simulink model "stewart_platform_model"  (R2020a)
settings: Solver=ode45  StartTime=0.0  StopTime=0.1  FixedStep=1e-4  MaxStep=0.2  RelTol=1e-4  AbsTol=1e-4
values from neighbouring files (symbols this model uses):
  ground = initializeGround('type', 'none')    [active_damping_dvf.m]    (also in active_damping_iff.m; active_damping_inertial.m; cubic_conf_coupling_cartesianl.m; cubic_conf_coupling_strutsl.m)
  payload = initializePayload('type', 'none')    [active_damping_dvf.m]    (also in active_damping_iff.m; active_damping_inertial.m; cubic_conf_coupling_cartesianl.m; cubic_conf_coupling_strutsl.m)
  s = zpk('s')    [active_damping_dvf.m]    (also in active_damping_iff.m; active_damping_inertial.m; cubic_conf_above_platforml.m; cubic_conf_coupling_cartesianl.m)
undefined symbols (not defined in the file or in its folder): X, Y, Z
libraries: sm_lib x29, nesl_utility x27, cstblocks x10
(part 1 of 2)
settings Model: Creator=thomas  LastModifiedBy=thomas
settings SolverCC: AutoScaleAbsTol=off
settings DataIOCC: SaveOutput=off  SignalLogging=off  DSMLogging=off  SaveTime=off  ReturnWorkspaceOutputs=off
settings DebuggingCC: SymbolicDimsDataTypeCodeGenerationDiagnostic=none
settings SFSimCC: CustomCodeUndefinedFunction=UseInterfaceOnly
settings SimscapeCC: SimscapeLogType=all  SimscapeLogSimulationStatistics=on  SimscapeLogDataHistory=10000
settings DiagnosticsConfigSet: SimMechanicsRigidlyBoundBlock=warning  SimMechanicsJointTargetOverSpecification=warning

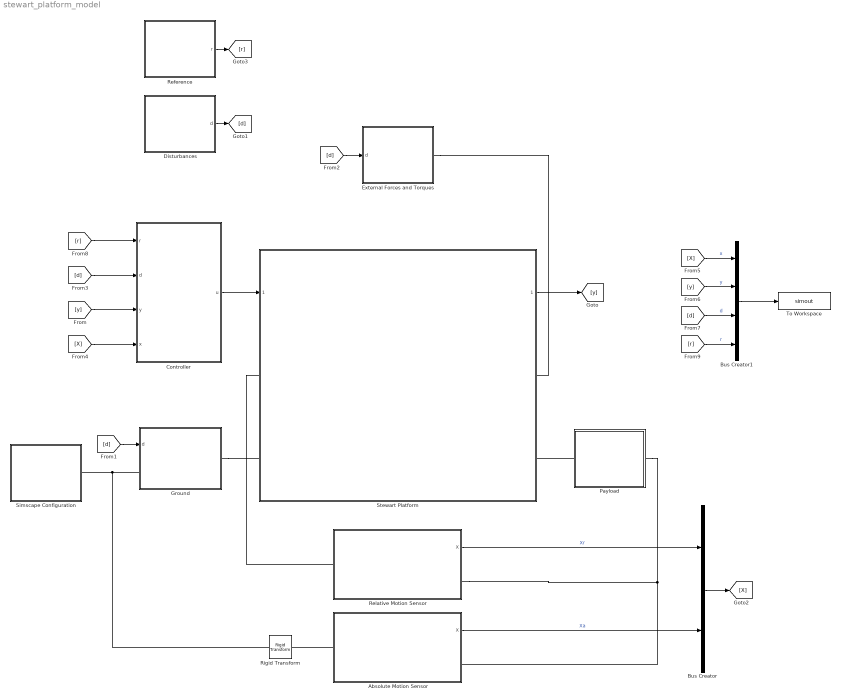
== system stewart_platform_model ==
  Absolute Motion Sensor : Subsystem
  Bus Creator : BusCreator  Inputs=2
  Bus Creator1 : BusCreator  Inputs=4
  Controller : Subsystem  Variant=on  VariantControl=Variant1
  Disturbances : Subsystem  VariantControl=disturbances.type == 1
  External Forces and Torques : Subsystem
  Ground : Subsystem  Variant=on  VariantControl=Variant1
  Payload : Subsystem  Variant=on  VariantControl=Variant1
  Reference : Subsystem  VariantControl=Variant1
  Relative Motion Sensor : Subsystem
  Rigid Transform : sm_lib/Frames and Transforms/Rigid Transform  TranslationMethod=Cartesian  TranslationStandardOffset=0  TranslationLengthUnit=m  TranslationStandardAxis=+Z  TranslationCartesianOffset=stewart.platform_F.FO_A  TranslationROffset=0  TranslationROffsetUnits=m  TranslationZOffset=0  TranslationZOffsetUnits=m  TranslationThetaOffset=0  TranslationThetaOffsetUnits=deg  RotationMethod=None  RotationAngleUnits=deg  RotationStandardAxis=+Z  RotationAngle=0.0  RotationArbitraryAxis=[0 0 1]  FollAlignAxisA=+X  BaseAlignAxisA=+Y  FollAlignAxisB=+Y  BaseAlignAxisB=+Z  RotationSequenceAxes=FollowerAxes  RotationSequence=XYX  RotationSequenceAngles=[0 0 0]  RotationSequenceAnglesUnits=deg  RotationMatrix=[1 0 0; 0 1 0; 0 0 1]
  Simscape Configuration : Subsystem
  Stewart Platform : Subsystem  ReferencedSubsystem=Stewart_Platform
  To Workspace : ToWorkspace  VariableName=simout  SaveFormat=Timeseries  SampleTime=-1
  wires:
  Stewart Platform/1 -> [y]
  Controller/1(u) -> Stewart Platform/1
  [d] -> Ground/1(d)
  [d] -> External Forces and Torques/1(d)
  Relative Motion Sensor/1(X) -> Bus Creator/1  "Xr"
  Absolute Motion Sensor/1(X) -> Bus Creator/2  "Xa"
  [y] -> Controller/3(y)
  [d] -> Controller/2(d)
  Bus Creator/1 -> [X]
  [X] -> Controller/4(x)
  Disturbances/1(d) -> [d]
  Bus Creator1/1 -> To Workspace/1
  [y] -> Bus Creator1/2  "y"
  [X] -> Bus Creator1/1  "x"
  [d] -> Bus Creator1/3  "d"
  Reference/1(r) -> [r]
  [r] -> Controller/1(r)
  [r] -> Bus Creator1/4  "r"
  connections:
  Ground/LConn1 -- Rigid Transform/LConn1 -- Simscape Configuration/RConn1
  Ground/RConn1 -- Stewart Platform/LConn2
  Payload/LConn1 -- Stewart Platform/RConn2
  External Forces and Torques/RConn1 -- Stewart Platform/RConn1
  Relative Motion Sensor/LConn1 -- Stewart Platform/LConn1
  Absolute Motion Sensor/LConn1 -- Rigid Transform/RConn1
  Relative Motion Sensor/RConn1 -- Payload/RConn1 -- Absolute Motion Sensor/RConn1

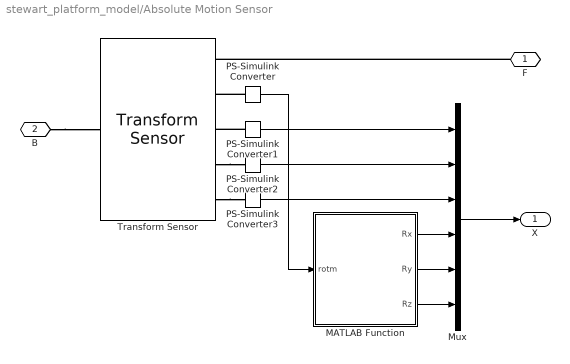
== system stewart_platform_model/Absolute Motion Sensor ==
  MATLAB Function : MATLAB Function  TreatAsAtomicUnit=on
  Mux : Mux  Inputs=6
  PS-Simulink Converter{,1..3} (4 alike) : nesl_utility/PS-Simulink Converter  PhysicalDomain=network_engine_domain  SubClassName=ps_output  LeftPortType=input  RightPortType=output  PseudoPeriodic=off  Frequencies=[]  Unit=inherit  AffineConversion=off
  Transform Sensor : sm_lib/Frames and Transforms/Transform Sensor  MeasurementFrame=Base  SenseAngle=off  SenseAxis=off  SenseAngle1=off  SenseAngle2=off  SenseAngle3=off  SenseQ=off  SenseR=on  SenseOmegaX=off  SenseOmegaY=off  SenseOmegaZ=off  SenseOmega1=off  SenseOmega2=off  SenseOmega3=off  SenseQDot=off  SenseRDot=off  SenseAlphaX=off  SenseAlphaY=off  SenseAlphaZ=off  SenseAlpha1=off  SenseAlpha2=off  SenseAlpha3=off  SenseQDDot=off  SenseRDDot=off  SenseX=on  SenseY=on  SenseZ=on  SenseRad=off  SenseAzim=off  SenseDist=off  SenseInc=off  SenseXDot=off  SenseYDot=off  SenseZDot=off  SenseRadDot=off  SenseAzimDot=off  SenseDistDot=off  SenseIncDot=off  SenseXDDot=off  SenseYDDot=off  SenseZDDot=off  SenseRadDDot=off  SenseAzimDDot=off  SenseDistDDot=off  SenseIncDDot=off
  F : PMIOPort  Side=Right
  B : PMIOPort  Port=2  Side=Left
  X : Outport
  wires:
  PS-Simulink Converter3/1 -> Mux/3
  MATLAB Function/1(Rx) -> Mux/4
  Mux/1 -> X/1
  MATLAB Function/2(Ry) -> Mux/5
  PS-Simulink Converter/1 -> MATLAB Function/1(rotm)
  MATLAB Function/3(Rz) -> Mux/6
  PS-Simulink Converter1/1 -> Mux/1
  PS-Simulink Converter2/1 -> Mux/2
  connections:
  PS-Simulink Converter1/LConn1 -- Transform Sensor/RConn3
  Transform Sensor/RConn4 -- PS-Simulink Converter2/LConn1
  F/RConn1 -- Transform Sensor/RConn1
  Transform Sensor/RConn5 -- PS-Simulink Converter3/LConn1
  PS-Simulink Converter/LConn1 -- Transform Sensor/RConn2
  B/RConn1 -- Transform Sensor/LConn1

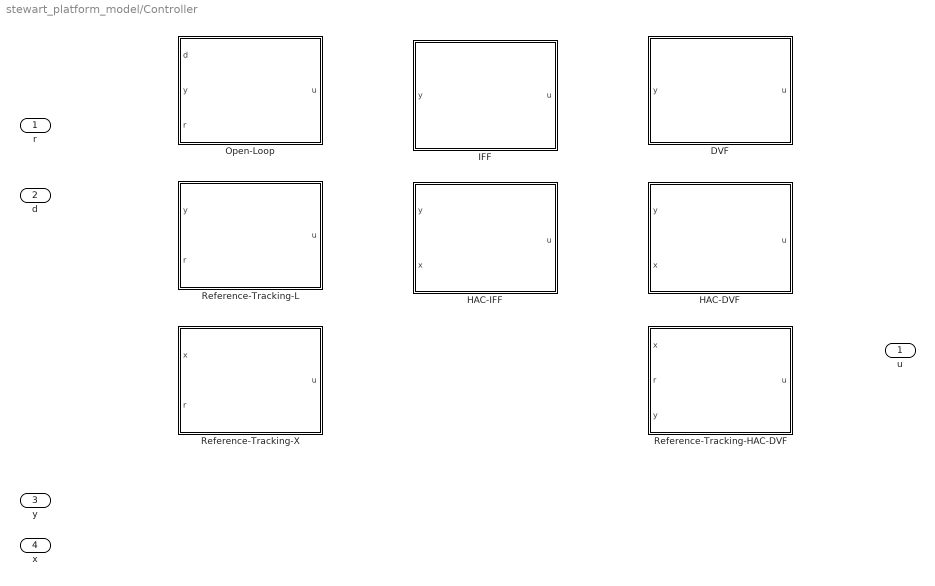
== system stewart_platform_model/Controller ==
  r : Inport
  d : Inport  Port=2
  y : Inport  Port=3
  x : Inport  Port=4
  DVF : Subsystem  VariantControl=controller.type == 2
  HAC-DVF : Subsystem  VariantControl=controller.type == 4
  HAC-IFF : Subsystem  VariantControl=controller.type == 3
  IFF : Subsystem  VariantControl=controller.type == 1
  Open-Loop : Subsystem  VariantControl=controller.type == 0
  Reference-Tracking-HAC-DVF : Subsystem  VariantControl=controller.type == 7
  Reference-Tracking-L : Subsystem  VariantControl=controller.type == 5
  Reference-Tracking-X : Subsystem  VariantControl=controller.type == 6
  u : Outport

== system stewart_platform_model/Disturbances ==
  Bus Creator : BusCreator  Inputs=2
  From Workspace : FromWorkspace  VariableName=disturbances.Fd  OutDataTypeStr=double  OutputAfterFinalValue=Setting to zero
  From Workspace1 : FromWorkspace  VariableName=disturbances.Dw  OutDataTypeStr=double  OutputAfterFinalValue=Setting to zero
  d : Outport
  wires:
  Bus Creator/1 -> d/1
  From Workspace/1 -> Bus Creator/1  "F_ext"
  From Workspace1/1 -> Bus Creator/2  "D_w"

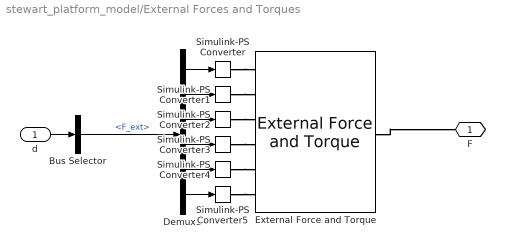
== system stewart_platform_model/External Forces and Torques ==
  d : Inport
  Bus Selector : BusSelector  OutputSignals=F_ext
  Demux1 : Demux  Outputs=6
  External Force and Torque : sm_lib/Forces and Torques/External Force and Torque  ForceResolutionFrame=World  EnableForceX=on  EnableForceY=on  EnableForceZ=on  EnableForce=off  TorqueResolutionFrame=World  EnableTorqueX=on  EnableTorqueY=on  EnableTorqueZ=on  EnableTorque=off
  Simulink-PS Converter{,1..5} (6 alike) : nesl_utility/Simulink-PS Converter  PhysicalDomain=network_engine_domain  SubClassName=ps_input  LeftPortType=input  RightPortType=output  PseudoPeriodic=off  Frequencies=[]  NoiseDistribution=none  NoiseParameters=[]  Unit=1  AffineConversion=off  FilteringAndDerivatives=provide  SimscapeFilterOrder=1  InputFilterTimeConstant=0.001  UdotUserProvided=0
  F : PMIOPort  Side=Right
  wires:
  Demux1/4 -> Simulink-PS Converter3/1
  Demux1/1 -> Simulink-PS Converter/1
  Demux1/6 -> Simulink-PS Converter5/1
  Demux1/2 -> Simulink-PS Converter1/1
  Demux1/5 -> Simulink-PS Converter4/1
  Demux1/3 -> Simulink-PS Converter2/1
  d/1 -> Bus Selector/1
  Bus Selector/1 -> Demux1/1  "<F_ext>"
  connections:
  Simulink-PS Converter1/RConn1 -- External Force and Torque/LConn2
  External Force and Torque/RConn1 -- F/RConn1
  Simulink-PS Converter2/RConn1 -- External Force and Torque/LConn3
  Simulink-PS Converter3/RConn1 -- External Force and Torque/LConn4
  Simulink-PS Converter5/RConn1 -- External Force and Torque/LConn6
  Simulink-PS Converter4/RConn1 -- External Force and Torque/LConn5
  Simulink-PS Converter/RConn1 -- External Force and Torque/LConn1

== system stewart_platform_model/Ground ==
  d : Inport
  Flexible : Subsystem  VariantControl=ground.type == 3
  None : Subsystem  VariantControl=ground.type == 1
  Rigid : Subsystem  VariantControl=ground.type == 2
  "{W}" : PMIOPort  Side=Left
  "{F}" : PMIOPort  Port=2  Side=Right

== system stewart_platform_model/Payload ==
  Cartesian : Subsystem  VariantControl=payload.type == 4
  Flexible : Subsystem  VariantControl=payload.type == 3
  None : Subsystem  VariantControl=payload.type == 1
  Rigid : Subsystem  VariantControl=payload.type == 2
  "{M}" : PMIOPort  Side=Left
  "{P}" : PMIOPort  Port=2  Side=Right

== system stewart_platform_model/Reference ==
  Bus Creator : BusCreator  Inputs=2
  From Workspace : FromWorkspace  VariableName=references.r  OutDataTypeStr=double  OutputAfterFinalValue=Setting to zero
  From Workspace1 : FromWorkspace  VariableName=references.rL  OutDataTypeStr=double  OutputAfterFinalValue=Setting to zero
  r : Outport
  wires:
  Bus Creator/1 -> r/1
  From Workspace1/1 -> Bus Creator/2  "rL"
  From Workspace/1 -> Bus Creator/1  "r"

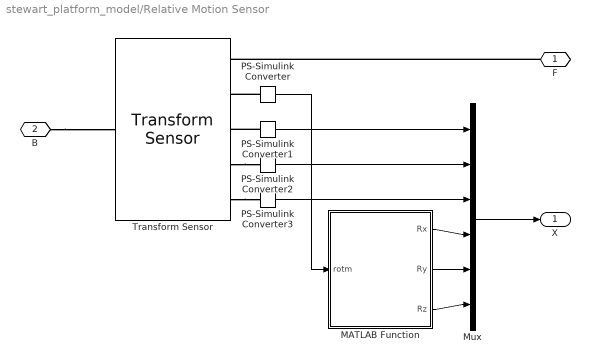
== system stewart_platform_model/Relative Motion Sensor ==
  MATLAB Function : MATLAB Function  TreatAsAtomicUnit=on
  Mux : Mux  Inputs=6
  PS-Simulink Converter{,1..3} (4 alike) : nesl_utility/PS-Simulink Converter  PhysicalDomain=network_engine_domain  SubClassName=ps_output  LeftPortType=input  RightPortType=output  PseudoPeriodic=off  Frequencies=[]  Unit=inherit  AffineConversion=off
  Transform Sensor : sm_lib/Frames and Transforms/Transform Sensor  MeasurementFrame=Base  SenseAngle=off  SenseAxis=off  SenseAngle1=off  SenseAngle2=off  SenseAngle3=off  SenseQ=off  SenseR=on  SenseOmegaX=off  SenseOmegaY=off  SenseOmegaZ=off  SenseOmega1=off  SenseOmega2=off  SenseOmega3=off  SenseQDot=off  SenseRDot=off  SenseAlphaX=off  SenseAlphaY=off  SenseAlphaZ=off  SenseAlpha1=off  SenseAlpha2=off  SenseAlpha3=off  SenseQDDot=off  SenseRDDot=off  SenseX=on  SenseY=on  SenseZ=on  SenseRad=off  SenseAzim=off  SenseDist=off  SenseInc=off  SenseXDot=off  SenseYDot=off  SenseZDot=off  SenseRadDot=off  SenseAzimDot=off  SenseDistDot=off  SenseIncDot=off  SenseXDDot=off  SenseYDDot=off  SenseZDDot=off  SenseRadDDot=off  SenseAzimDDot=off  SenseDistDDot=off  SenseIncDDot=off
  F : PMIOPort  Side=Right
  B : PMIOPort  Port=2  Side=Left
  X : Outport
  wires:
  PS-Simulink Converter/1 -> MATLAB Function/1(rotm)
  MATLAB Function/3(Rz) -> Mux/6
  MATLAB Function/1(Rx) -> Mux/4
  MATLAB Function/2(Ry) -> Mux/5
  PS-Simulink Converter3/1 -> Mux/3
  PS-Simulink Converter2/1 -> Mux/2
  PS-Simulink Converter1/1 -> Mux/1
  Mux/1 -> X/1
  connections:
  B/RConn1 -- Transform Sensor/LConn1
  F/RConn1 -- Transform Sensor/RConn1
  PS-Simulink Converter/LConn1 -- Transform Sensor/RConn2
  PS-Simulink Converter1/LConn1 -- Transform Sensor/RConn3
  Transform Sensor/RConn4 -- PS-Simulink Converter2/LConn1
  Transform Sensor/RConn5 -- PS-Simulink Converter3/LConn1

== system stewart_platform_model/Simscape Configuration ==
  Mechanism Configuration : sm_lib/Utilities/Mechanism Configuration  UniformGravity=None  GravityVector=[0 0 -9.8]  GravityUnits=m/s^2  LinearizationDelta=1e-8
  Solver Configuration : nesl_utility/Solver Configuration  PhysicalDomain=network_engine_domain  SubClassName=solver  LeftPortType=input  RightPortType=generic  Tones=[]  Harmonics=[]  SimulateNoise=off  Profile=off  UseLocalSampling=off  EnableSwitchedLinearOptims=on  FrequencyDomain=off  UseCCode=off  RelTol=0.001  AbsTol=1e-06  MinStep=1e-09  ToWorkspace=off  RevertToSquareIcSolve=off  NumHomotopyIterations=100  PhasorMode=off  PhasorModeNumHarmonics=1  DoDC=off  ResidualTolerance=1e-09  UseLocalSolver=off  LocalSolverChoice=NE_BACKWARD_EULER_ADVANCER  LocalSolverSampleTime=0.001  DoFixedCost=off  MaxNonlinIter=3  MaxModeIter=2  LinearAlgebra=auto  EquationFormulation=NE_TIME_EF  DelaysMemoryBudget=1024  AutomaticFiltering=off  FilteringTimeConstant=0.001  PartitionStorageMethod=AS_NEEDED  PartitionMemoryBudget=1024  PartitionMethod=ROBUST
  World Frame : sm_lib/Frames and Transforms/World Frame
  "{W}" : PMIOPort  Side=Right
  connections:
  World Frame/RConn1 -- "{W}"/RConn1 -- Solver Configuration/RConn1 -- Mechanism Configuration/RConn1

== system stewart_platform_model/Controller/DVF ==
  y : Inport
  Bus Selector : BusSelector  OutputSignals=dLm
  LTI System : cstblocks/LTI System  sys=K_dvf  IC=[]
  u : Outport
  wires:
  Bus Selector/1 -> LTI System/1  "<dLm>"
  y/1 -> Bus Selector/1
  LTI System/1 -> u/1

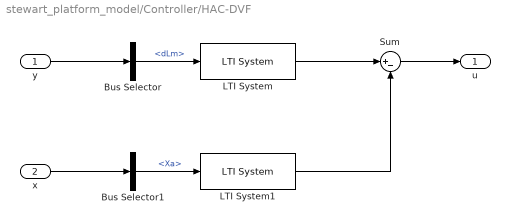
== system stewart_platform_model/Controller/HAC-DVF ==
  y : Inport
  x : Inport  Port=2
  Bus Selector : BusSelector  OutputSignals=dLm
  Bus Selector1 : BusSelector  OutputSignals=Xa
  LTI System : cstblocks/LTI System  sys=K_dvf  IC=[]
  LTI System1 : cstblocks/LTI System  sys=K_hac_dvf  IC=[]
  Sum : Sum  Inputs=|+-
  u : Outport
  wires:
  LTI System/1 -> Sum/1
  y/1 -> Bus Selector/1
  Bus Selector/1 -> LTI System/1  "<dLm>"
  x/1 -> Bus Selector1/1
  Bus Selector1/1 -> LTI System1/1  "<Xa>"
  Sum/1 -> u/1
  LTI System1/1 -> Sum/2

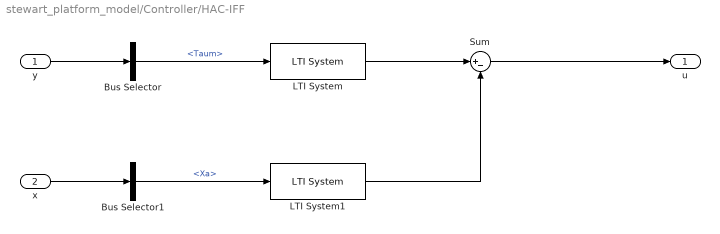
== system stewart_platform_model/Controller/HAC-IFF ==
  y : Inport
  x : Inport  Port=2
  Bus Selector : BusSelector  OutputSignals=Taum
  Bus Selector1 : BusSelector  OutputSignals=Xa
  LTI System : cstblocks/LTI System  sys=K_iff  IC=[]
  LTI System1 : cstblocks/LTI System  sys=K_hac_iff  IC=[]
  Sum : Sum  Inputs=|+-
  u : Outport
  wires:
  x/1 -> Bus Selector1/1
  Bus Selector/1 -> LTI System/1  "<Taum>"
  LTI System1/1 -> Sum/2
  y/1 -> Bus Selector/1
  Sum/1 -> u/1
  Bus Selector1/1 -> LTI System1/1  "<Xa>"
  LTI System/1 -> Sum/1

== system stewart_platform_model/Controller/IFF ==
  y : Inport
  Bus Selector : BusSelector  OutputSignals=Taum
  LTI System : cstblocks/LTI System  sys=K_iff  IC=[]
  u : Outport
  wires:
  LTI System/1 -> u/1
  y/1 -> Bus Selector/1
  Bus Selector/1 -> LTI System/1  "<Taum>"

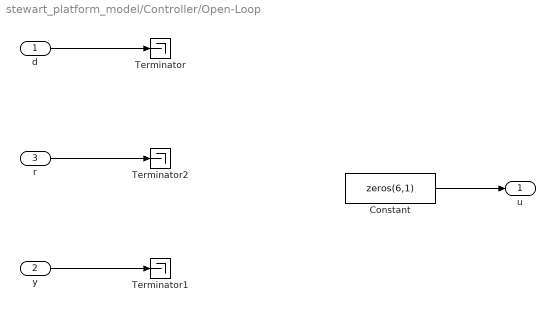
== system stewart_platform_model/Controller/Open-Loop ==
  d : Inport
  y : Inport  Port=2
  r : Inport  Port=3
  Constant : Constant  Value=zeros(6,1)
  Terminator : Terminator
  Terminator1 : Terminator
  Terminator2 : Terminator
  u : Outport
  wires:
  y/1 -> Terminator1/1
  Constant/1 -> u/1
  d/1 -> Terminator/1
  r/1 -> Terminator2/1

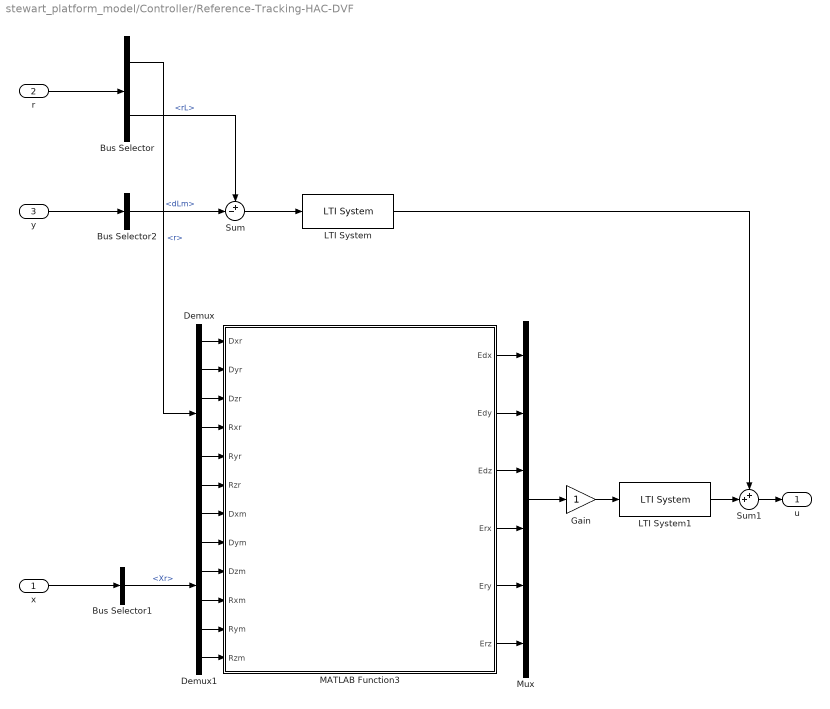
== system stewart_platform_model/Controller/Reference-Tracking-HAC-DVF ==
  x : Inport
  r : Inport  Port=2
  y : Inport  Port=3
  Bus Selector : BusSelector  OutputSignals=r,rL
  Bus Selector1 : BusSelector  OutputSignals=Xr
  Bus Selector2 : BusSelector  OutputSignals=dLm
  Demux : Demux  Outputs=6
  Demux1 : Demux  Outputs=6
  Gain : Gain
  LTI System : cstblocks/LTI System  sys=Kl  IC=[]
  LTI System1 : cstblocks/LTI System  sys=Kx  IC=[]
  MATLAB Function3 : MATLAB Function  TreatAsAtomicUnit=on
  Mux : Mux  Inputs=6
  Sum : Sum  Inputs=+-|
  Sum1 : Sum  Inputs=++|
  u : Outport
  wires:
  MATLAB Function3/6(Erz) -> Mux/6
  MATLAB Function3/5(Ery) -> Mux/5
  MATLAB Function3/4(Erx) -> Mux/4
  MATLAB Function3/3(Edz) -> Mux/3
  MATLAB Function3/2(Edy) -> Mux/2
  MATLAB Function3/1(Edx) -> Mux/1
  Demux1/6 -> MATLAB Function3/12(Rzm)
  Demux1/5 -> MATLAB Function3/11(Rym)
  Demux1/4 -> MATLAB Function3/10(Rxm)
  Demux1/3 -> MATLAB Function3/9(Dzm)
  Demux1/2 -> MATLAB Function3/8(Dym)
  Demux1/1 -> MATLAB Function3/7(Dxm)
  Demux/6 -> MATLAB Function3/6(Rzr)
  Demux/5 -> MATLAB Function3/5(Ryr)
  Demux/4 -> MATLAB Function3/4(Rxr)
  Demux/3 -> MATLAB Function3/3(Dzr)
  Demux/2 -> MATLAB Function3/2(Dyr)
  Demux/1 -> MATLAB Function3/1(Dxr)
  Mux/1 -> Gain/1
  x/1 -> Bus Selector1/1
  r/1 -> Bus Selector/1
  y/1 -> Bus Selector2/1
  Bus Selector/2 -> Sum/1  "<rL>"
  Bus Selector2/1 -> Sum/2  "<dLm>"
  Sum/1 -> LTI System/1
  Bus Selector1/1 -> Demux1/1  "<Xr>"
  Bus Selector/1 -> Demux/1  "<r>"
  Gain/1 -> LTI System1/1
  Sum1/1 -> u/1
  LTI System1/1 -> Sum1/2
  LTI System/1 -> Sum1/1

== system stewart_platform_model/Controller/Reference-Tracking-L ==
  y : Inport
  r : Inport  Port=2
  Bus Selector : BusSelector  OutputSignals=rL
  Bus Selector1 : BusSelector  OutputSignals=dLm
  LTI System : cstblocks/LTI System  sys=Kl  IC=[]
  Sum : Sum  Inputs=|+-
  u : Outport
  wires:
  LTI System/1 -> u/1
  y/1 -> Bus Selector1/1
  r/1 -> Bus Selector/1
  Bus Selector/1 -> Sum/1  "<rL>"
  Bus Selector1/1 -> Sum/2  "<dLm>"
  Sum/1 -> LTI System/1

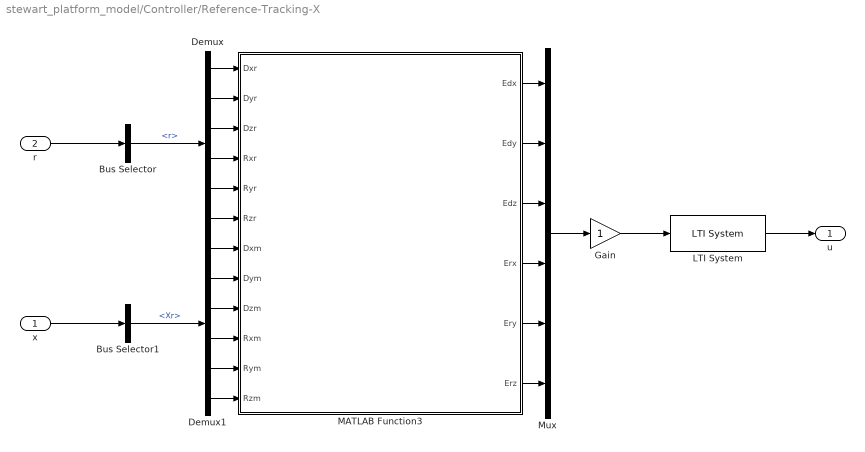
== system stewart_platform_model/Controller/Reference-Tracking-X ==
  x : Inport
  r : Inport  Port=2
  Bus Selector : BusSelector  OutputSignals=r
  Bus Selector1 : BusSelector  OutputSignals=Xr
  Demux : Demux  Outputs=6
  Demux1 : Demux  Outputs=6
  Gain : Gain
  LTI System : cstblocks/LTI System  sys=K  IC=[]
  MATLAB Function3 : MATLAB Function  TreatAsAtomicUnit=on
  Mux : Mux  Inputs=6
  u : Outport
  wires:
  r/1 -> Bus Selector/1
  x/1 -> Bus Selector1/1
  Bus Selector1/1 -> Demux1/1  "<Xr>"
  Mux/1 -> Gain/1
  LTI System/1 -> u/1
  Bus Selector/1 -> Demux/1  "<r>"
  Gain/1 -> LTI System/1
  Demux/1 -> MATLAB Function3/1(Dxr)
  Demux/2 -> MATLAB Function3/2(Dyr)
  Demux/3 -> MATLAB Function3/3(Dzr)
  Demux/4 -> MATLAB Function3/4(Rxr)
  Demux/5 -> MATLAB Function3/5(Ryr)
  Demux/6 -> MATLAB Function3/6(Rzr)
  Demux1/1 -> MATLAB Function3/7(Dxm)
  Demux1/2 -> MATLAB Function3/8(Dym)
  Demux1/3 -> MATLAB Function3/9(Dzm)
  Demux1/4 -> MATLAB Function3/10(Rxm)
  Demux1/5 -> MATLAB Function3/11(Rym)
  Demux1/6 -> MATLAB Function3/12(Rzm)
  MATLAB Function3/1(Edx) -> Mux/1
  MATLAB Function3/2(Edy) -> Mux/2
  MATLAB Function3/3(Edz) -> Mux/3
  MATLAB Function3/4(Erx) -> Mux/4
  MATLAB Function3/5(Ery) -> Mux/5
  MATLAB Function3/6(Erz) -> Mux/6

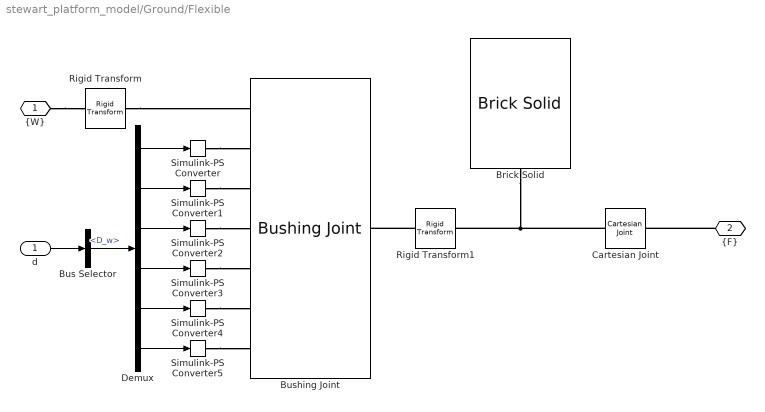
== system stewart_platform_model/Ground/Flexible ==
  d : Inport
  Brick Solid : sm_lib/Body Elements/Brick Solid  GraphicAmbientColor=[0.15 0.15 0.15 1.0]  BasedOnType=Density  BrickDimensions=[0.5 0.5 0.1]  BrickDimensionUnits=m  CenterOfMass=[0 0 0]  CenterOfMassUnits=m  GraphicDiffuseColor=[0.5 0.5 0.5]  Density=1000  DensityUnits=kg/m^3  DoExposeReferenceFrame=off  GraphicEmissiveColor=[0.0 0.0 0.0 1.0]  ExportEntireGeometry=off  SerializedFrames=<Frames><Frame><Id>Frame2</Id><Value><Name>top</Name><Origin><Source>GeometricFeature</Source><FeatureName>+z surface</FeatureName></Origin><PrimaryAxis><DefinedDirection>+Z</DefinedDirection><Source>ReferenceFrame</Source><SourceDirection>+Z</SourceDirection><FeatureName></FeatureName></PrimaryAxis><SecondaryAxis><DefinedDirection>+X</DefinedDirection><Source>ReferenceFrame</Source><SourceDirection>+X</SourceDirection><FeatureName></FeatureName></SecondaryAxis></Value></Frame></Frames>  MarkerShape=Sphere  MarkerSize=10  GraphicType=FromGeometry  InertiaType=CalculateFromGeometry  Mass=1  MassUnits=kg  MomentsOfInertia=[1 1 1]  MomentsOfInertiaUnits=kg*m^2  GraphicOpacity=1.0  ProductsOfInertia=[0 0 0]  ProductsOfInertiaUnits=kg*m^2  GraphicShininess=75  GraphicSpecularColor=[0.5 0.5 0.5 1.0]  GraphicVisPropType=SimpleVisualProperties
  Bus Selector : BusSelector  OutputSignals=D_w
  Bushing Joint : sm_lib/Joints/Bushing Joint  JointMode=Normal  SenseConstraintForce=off  SenseConstraintForceX=off  SenseConstraintForceY=off  SenseConstraintForceZ=off  SenseConstraintTorque=off  SenseConstraintTorqueX=off  SenseConstraintTorqueY=off  SenseConstraintTorqueZ=off  SenseTotalForce=off  SenseTotalForceX=off  SenseTotalForceY=off  SenseTotalForceZ=off  SenseTotalTorque=off  SenseTotalTorqueX=off  SenseTotalTorqueY=off  SenseTotalTorqueZ=off  CompositeWrenchDir=FollowerOnBase  CompositeWrenchFrame=BaseFrame  PxEquilibriumPosition=0  PxEquilibriumPositionUnits=m  PxSpringStiffness=0  PxSpringStiffnessUnits=N/m  PxDampingCoefficient=0  PxDampingCoefficientUnits=N/(m/s)  PxTorqueActuationMode=ComputedTorque  PxMotionActuationMode=InputMotion  PxSensePosition=off  PxSenseVelocity=off  PxSenseAcceleration=off  PxSenseTorqueForce=off  PxSenseLowerLimitTorqueForce=off  PxSenseUpperLimitTorqueForce=off  PxLowerLimitSpecify=off  PxLowerLimitBound=-1  PxLowerLimitBoundUnits=m  PxLowerLimitStiffness=1e6  PxLowerLimitStiffnessUnits=N/m  PxLowerLimitDamping=1e3  PxLowerLimitDampingUnits=N/(m/s)  PxLowerLimitTransitionRegionWidth=1e-4  PxLowerLimitTransitionRegionWidthUnits=m  PxUpperLimitSpecify=off  PxUpperLimitBound=1  PxUpperLimitBoundUnits=m  PxUpperLimitStiffness=1e6  PxUpperLimitStiffnessUnits=N/m  PxUpperLimitDamping=1e3  PxUpperLimitDampingUnits=N/(m/s)  PxUpperLimitTransitionRegionWidth=1e-4  PxUpperLimitTransitionRegionWidthUnits=m  PxPositionTargetSpecify=off  PxPositionTargetPriority=High  PxPositionTargetValue=0  PxPositionTargetValueUnits=m  PxVelocityTargetSpecify=off  PxVelocityTargetPriority=High  PxVelocityTargetValue=0  PxVelocityTargetValueUnits=m/s  PyEquilibriumPosition=0  PyEquilibriumPositionUnits=m  PySpringStiffness=0  PySpringStiffnessUnits=N/m  PyDampingCoefficient=0  PyDampingCoefficientUnits=N/(m/s)  PyTorqueActuationMode=ComputedTorque  PyMotionActuationMode=InputMotion  PySensePosition=off  PySenseVelocity=off  PySenseAcceleration=off  PySenseTorqueForce=off  PySenseLowerLimitTorqueForce=off  PySenseUpperLimitTorqueForce=off  PyLowerLimitSpecify=off  PyLowerLimitBound=-1  PyLowerLimitBoundUnits=m  PyLowerLimitStiffness=1e6  PyLowerLimitStiffnessUnits=N/m  PyLowerLimitDamping=1e3  PyLowerLimitDampingUnits=N/(m/s)  PyLowerLimitTransitionRegionWidth=1e-4  PyLowerLimitTransitionRegionWidthUnits=m  PyUpperLimitSpecify=off  PyUpperLimitBound=1  PyUpperLimitBoundUnits=m  PyUpperLimitStiffness=1e6  PyUpperLimitStiffnessUnits=N/m  PyUpperLimitDamping=1e3  PyUpperLimitDampingUnits=N/(m/s)  PyUpperLimitTransitionRegionWidth=1e-4  PyUpperLimitTransitionRegionWidthUnits=m  PyPositionTargetSpecify=off  PyPositionTargetPriority=High  PyPositionTargetValue=0  PyPositionTargetValueUnits=m  PyVelocityTargetSpecify=off  PyVelocityTargetPriority=High  PyVelocityTargetValue=0  PyVelocityTargetValueUnits=m/s  PzEquilibriumPosition=0  PzEquilibriumPositionUnits=m  PzSpringStiffness=0  PzSpringStiffnessUnits=N/m  PzDampingCoefficient=0  PzDampingCoefficientUnits=N/(m/s)  PzTorqueActuationMode=ComputedTorque  PzMotionActuationMode=InputMotion  PzSensePosition=off  PzSenseVelocity=off  PzSenseAcceleration=off  PzSenseTorqueForce=off  PzSenseLowerLimitTorqueForce=off  PzSenseUpperLimitTorqueForce=off  PzLowerLimitSpecify=off  PzLowerLimitBound=-1  PzLowerLimitBoundUnits=m  PzLowerLimitStiffness=1e6  PzLowerLimitStiffnessUnits=N/m  PzLowerLimitDamping=1e3  PzLowerLimitDampingUnits=N/(m/s)  PzLowerLimitTransitionRegionWidth=1e-4  PzLowerLimitTransitionRegionWidthUnits=m  PzUpperLimitSpecify=off  PzUpperLimitBound=1  PzUpperLimitBoundUnits=m  PzUpperLimitStiffness=1e6  PzUpperLimitStiffnessUnits=N/m  PzUpperLimitDamping=1e3  PzUpperLimitDampingUnits=N/(m/s)  PzUpperLimitTransitionRegionWidth=1e-4  PzUpperLimitTransitionRegionWidthUnits=m  PzPositionTargetSpecify=off  PzPositionTargetPriority=High  PzPositionTargetValue=0  PzPositionTargetValueUnits=m  PzVelocityTargetSpecify=off  PzVelocityTargetPriority=High  PzVelocityTargetValue=0  PzVelocityTargetValueUnits=m/s  RxEquilibriumPosition=0  RxEquilibriumPositionUnits=deg  RxSpringStiffness=0  RxSpringStiffnessUnits=N*m/deg  RxDampingCoefficient=0  RxDampingCoefficientUnits=N*m/(deg/s)  RxTorqueActuationMode=ComputedTorque  RxMotionActuationMode=InputMotion  RxSensePosition=off  RxSenseVelocity=off  RxSenseAcceleration=off  RxSenseTorqueForce=off  RxSenseLowerLimitTorqueForce=off  RxSenseUpperLimitTorqueForce=off  RxLowerLimitSpecify=off  RxLowerLimitBound=-90  RxLowerLimitBoundUnits=deg  RxLowerLimitStiffness=1e4  RxLowerLimitStiffnessUnits=N*m/deg  RxLowerLimitDamping=10  RxLowerLimitDampingUnits=N*m/(deg/s)  RxLowerLimitTransitionRegionWidth=0.1  RxLowerLimitTransitionRegionWidthUnits=deg  RxUpperLimitSpecify=off  RxUpperLimitBound=90  RxUpperLimitBoundUnits=deg  RxUpperLimitStiffness=1e4  RxUpperLimitStiffnessUnits=N*m/deg  RxUpperLimitDamping=10  RxUpperLimitDampingUnits=N*m/(deg/s)  RxUpperLimitTransitionRegionWidth=0.1  RxUpperLimitTransitionRegionWidthUnits=deg  RxPositionTargetSpecify=off  RxPositionTargetPriority=High  RxPositionTargetValue=0  RxPositionTargetValueUnits=deg  RxVelocityTargetSpecify=off  RxVelocityTargetPriority=High  RxVelocityTargetValue=0  RxVelocityTargetValueUnits=deg/s  RyEquilibriumPosition=0  RyEquilibriumPositionUnits=deg  RySpringStiffness=0  RySpringStiffnessUnits=N*m/deg  RyDampingCoefficient=0  RyDampingCoefficientUnits=N*m/(deg/s)  RyTorqueActuationMode=ComputedTorque  RyMotionActuationMode=InputMotion  RySensePosition=off  RySenseVelocity=off  RySenseAcceleration=off  RySenseTorqueForce=off  RySenseLowerLimitTorqueForce=off  RySenseUpperLimitTorqueForce=off  RyLowerLimitSpecify=off  RyLowerLimitBound=-90  RyLowerLimitBoundUnits=deg  RyLowerLimitStiffness=1e4  RyLowerLimitStiffnessUnits=N*m/deg  RyLowerLimitDamping=10  RyLowerLimitDampingUnits=N*m/(deg/s)  RyLowerLimitTransitionRegionWidth=0.1  RyLowerLimitTransitionRegionWidthUnits=deg  RyUpperLimitSpecify=off  RyUpperLimitBound=90  RyUpperLimitBoundUnits=deg  RyUpperLimitStiffness=1e4  RyUpperLimitStiffnessUnits=N*m/deg  RyUpperLimitDamping=10  RyUpperLimitDampingUnits=N*m/(deg/s)  RyUpperLimitTransitionRegionWidth=0.1  RyUpperLimitTransitionRegionWidthUnits=deg  RyPositionTargetSpecify=off  RyPositionTargetPriority=High  RyPositionTargetValue=0  RyPositionTargetValueUnits=deg  RyVelocityTargetSpecify=off  RyVelocityTargetPriority=High  RyVelocityTargetValue=0  RyVelocityTargetValueUnits=deg/s  RzEquilibriumPosition=0  RzEquilibriumPositionUnits=deg  RzSpringStiffness=0  RzSpringStiffnessUnits=N*m/deg  RzDampingCoefficient=0  RzDampingCoefficientUnits=N*m/(deg/s)  RzTorqueActuationMode=ComputedTorque  RzMotionActuationMode=InputMotion  RzSensePosition=off  RzSenseVelocity=off  RzSenseAcceleration=off  RzSenseTorqueForce=off  RzSenseLowerLimitTorqueForce=off  RzSenseUpperLimitTorqueForce=off  RzLowerLimitSpecify=off  RzLowerLimitBound=-90  RzLowerLimitBoundUnits=deg  RzLowerLimitStiffness=1e4  RzLowerLimitStiffnessUnits=N*m/deg  RzLowerLimitDamping=10  RzLowerLimitDampingUnits=N*m/(deg/s)  RzLowerLimitTransitionRegionWidth=0.1  RzLowerLimitTransitionRegionWidthUnits=deg  RzUpperLimitSpecify=off  RzUpperLimitBound=90  RzUpperLimitBoundUnits=deg  RzUpperLimitStiffness=1e4  RzUpperLimitStiffnessUnits=N*m/deg  RzUpperLimitDamping=10  RzUpperLimitDampingUnits=N*m/(deg/s)  RzUpperLimitTransitionRegionWidth=0.1  RzUpperLimitTransitionRegionWidthUnits=deg  RzPositionTargetSpecify=off  RzPositionTargetPriority=High  RzPositionTargetValue=0  RzPositionTargetValueUnits=deg  RzVelocityTargetSpecify=off  RzVelocityTargetPriority=High  RzVelocityTargetValue=0  RzVelocityTargetValueUnits=deg/s
  Cartesian Joint : sm_lib/Joints/Cartesian Joint  JointMode=Normal  SenseConstraintForce=off  SenseConstraintForceX=off  SenseConstraintForceY=off  SenseConstraintForceZ=off  SenseConstraintTorque=off  SenseConstraintTorqueX=off  SenseConstraintTorqueY=off  SenseConstraintTorqueZ=off  SenseTotalForce=off  SenseTotalForceX=off  SenseTotalForceY=off  SenseTotalForceZ=off  SenseTotalTorque=off  SenseTotalTorqueX=off  SenseTotalTorqueY=off  SenseTotalTorqueZ=off  CompositeWrenchDir=FollowerOnBase  CompositeWrenchFrame=BaseFrame  PxEquilibriumPosition=0  PxEquilibriumPositionUnits=m  PxSpringStiffness=ground.K(1)  PxSpringStiffnessUnits=N/m  PxDampingCoefficient=ground.C(1)  PxDampingCoefficientUnits=N/(m/s)  PxTorqueActuationMode=NoTorque  PxMotionActuationMode=ComputedMotion  PxSensePosition=off  PxSenseVelocity=off  PxSenseAcceleration=off  PxSenseTorqueForce=off  PxSenseLowerLimitTorqueForce=off  PxSenseUpperLimitTorqueForce=off  PxLowerLimitSpecify=off  PxLowerLimitBound=-1  PxLowerLimitBoundUnits=m  PxLowerLimitStiffness=1e6  PxLowerLimitStiffnessUnits=N/m  PxLowerLimitDamping=1e3  PxLowerLimitDampingUnits=N/(m/s)  PxLowerLimitTransitionRegionWidth=1e-4  PxLowerLimitTransitionRegionWidthUnits=m  PxUpperLimitSpecify=off  PxUpperLimitBound=1  PxUpperLimitBoundUnits=m  PxUpperLimitStiffness=1e6  PxUpperLimitStiffnessUnits=N/m  PxUpperLimitDamping=1e3  PxUpperLimitDampingUnits=N/(m/s)  PxUpperLimitTransitionRegionWidth=1e-4  PxUpperLimitTransitionRegionWidthUnits=m  PxPositionTargetSpecify=off  PxPositionTargetPriority=High  PxPositionTargetValue=0  PxPositionTargetValueUnits=m  PxVelocityTargetSpecify=off  PxVelocityTargetPriority=High  PxVelocityTargetValue=0  PxVelocityTargetValueUnits=m/s  PyEquilibriumPosition=0  PyEquilibriumPositionUnits=m  PySpringStiffness=ground.K(2)  PySpringStiffnessUnits=N/m  PyDampingCoefficient=ground.C(2)  PyDampingCoefficientUnits=N/(m/s)  PyTorqueActuationMode=NoTorque  PyMotionActuationMode=ComputedMotion  PySensePosition=off  PySenseVelocity=off  PySenseAcceleration=off  PySenseTorqueForce=off  PySenseLowerLimitTorqueForce=off  PySenseUpperLimitTorqueForce=off  PyLowerLimitSpecify=off  PyLowerLimitBound=-1  PyLowerLimitBoundUnits=m  PyLowerLimitStiffness=1e6  PyLowerLimitStiffnessUnits=N/m  PyLowerLimitDamping=1e3  PyLowerLimitDampingUnits=N/(m/s)  PyLowerLimitTransitionRegionWidth=1e-4  PyLowerLimitTransitionRegionWidthUnits=m  PyUpperLimitSpecify=off  PyUpperLimitBound=1  PyUpperLimitBoundUnits=m  PyUpperLimitStiffness=1e6  PyUpperLimitStiffnessUnits=N/m  PyUpperLimitDamping=1e3  PyUpperLimitDampingUnits=N/(m/s)  PyUpperLimitTransitionRegionWidth=1e-4  PyUpperLimitTransitionRegionWidthUnits=m  PyPositionTargetSpecify=off  PyPositionTargetPriority=High  PyPositionTargetValue=0  PyPositionTargetValueUnits=m  PyVelocityTargetSpecify=off  PyVelocityTargetPriority=High  PyVelocityTargetValue=0  PyVelocityTargetValueUnits=m/s  PzEquilibriumPosition=0  PzEquilibriumPositionUnits=m  PzSpringStiffness=ground.K(3)  PzSpringStiffnessUnits=N/m  PzDampingCoefficient=ground.C(3)  PzDampingCoefficientUnits=N/(m/s)  PzTorqueActuationMode=NoTorque  PzMotionActuationMode=ComputedMotion  PzSensePosition=off  PzSenseVelocity=off  PzSenseAcceleration=off  PzSenseTorqueForce=off  PzSenseLowerLimitTorqueForce=off  PzSenseUpperLimitTorqueForce=off  PzLowerLimitSpecify=off  PzLowerLimitBound=-1  PzLowerLimitBoundUnits=m  PzLowerLimitStiffness=1e6  PzLowerLimitStiffnessUnits=N/m  PzLowerLimitDamping=1e3  PzLowerLimitDampingUnits=N/(m/s)  PzLowerLimitTransitionRegionWidth=1e-4  PzLowerLimitTransitionRegionWidthUnits=m  PzUpperLimitSpecify=off  PzUpperLimitBound=1  PzUpperLimitBoundUnits=m  PzUpperLimitStiffness=1e6  PzUpperLimitStiffnessUnits=N/m  PzUpperLimitDamping=1e3  PzUpperLimitDampingUnits=N/(m/s)  PzUpperLimitTransitionRegionWidth=1e-4  PzUpperLimitTransitionRegionWidthUnits=m  PzPositionTargetSpecify=off  PzPositionTargetPriority=High  PzPositionTargetValue=0  PzPositionTargetValueUnits=m  PzVelocityTargetSpecify=off  PzVelocityTargetPriority=High  PzVelocityTargetValue=0  PzVelocityTargetValueUnits=m/s
  Demux : Demux  Outputs=6
  Rigid Transform : sm_lib/Frames and Transforms/Rigid Transform  TranslationMethod=Cartesian  TranslationStandardOffset=0  TranslationLengthUnit=m  TranslationStandardAxis=+Z  TranslationCartesianOffset=ground.rot_point  TranslationROffset=0  TranslationROffsetUnits=m  TranslationZOffset=0  TranslationZOffsetUnits=m  TranslationThetaOffset=0  TranslationThetaOffsetUnits=deg  RotationMethod=None  RotationAngleUnits=deg  RotationStandardAxis=+Z  RotationAngle=0.0  RotationArbitraryAxis=[0 0 1]  FollAlignAxisA=+X  BaseAlignAxisA=+Y  FollAlignAxisB=+Y  BaseAlignAxisB=+Z  RotationSequenceAxes=FollowerAxes  RotationSequence=XYX  RotationSequenceAngles=[0 0 0]  RotationSequenceAnglesUnits=deg  RotationMatrix=[1 0 0; 0 1 0; 0 0 1]
  Rigid Transform1 : sm_lib/Frames and Transforms/Rigid Transform  TranslationMethod=Cartesian  TranslationStandardOffset=0  TranslationLengthUnit=m  TranslationStandardAxis=+Z  TranslationCartesianOffset=ground.rot_point  TranslationROffset=0  TranslationROffsetUnits=m  TranslationZOffset=0  TranslationZOffsetUnits=m  TranslationThetaOffset=0  TranslationThetaOffsetUnits=deg  RotationMethod=None  RotationAngleUnits=deg  RotationStandardAxis=+Z  RotationAngle=0.0  RotationArbitraryAxis=[0 0 1]  FollAlignAxisA=+X  BaseAlignAxisA=+Y  FollAlignAxisB=+Y  BaseAlignAxisB=+Z  RotationSequenceAxes=FollowerAxes  RotationSequence=XYX  RotationSequenceAngles=[0 0 0]  RotationSequenceAnglesUnits=deg  RotationMatrix=[1 0 0; 0 1 0; 0 0 1]
  Simulink-PS Converter{,1..5} (6 alike) : nesl_utility/Simulink-PS Converter  PhysicalDomain=network_engine_domain  SubClassName=ps_input  LeftPortType=input  RightPortType=output  PseudoPeriodic=off  Frequencies=[]  NoiseDistribution=none  NoiseParameters=[]  Unit=1  AffineConversion=off  FilteringAndDerivatives=filter  SimscapeFilterOrder=2  InputFilterTimeConstant=0.001  UdotUserProvided=0
  "{W}" : PMIOPort  Side=Left
  "{F}" : PMIOPort  Port=2  Side=Right
  wires:
  Demux/3 -> Simulink-PS Converter2/1
  Bus Selector/1 -> Demux/1  "<D_w>"
  Demux/4 -> Simulink-PS Converter3/1
  Demux/2 -> Simulink-PS Converter1/1
  Demux/6 -> Simulink-PS Converter5/1
  Demux/5 -> Simulink-PS Converter4/1
  d/1 -> Bus Selector/1
  Demux/1 -> Simulink-PS Converter/1
  connections:
  Simulink-PS Converter1/RConn1 -- Bushing Joint/LConn3
  Simulink-PS Converter3/RConn1 -- Bushing Joint/LConn5
  Simulink-PS Converter2/RConn1 -- Bushing Joint/LConn4
  Simulink-PS Converter5/RConn1 -- Bushing Joint/LConn7
  Rigid Transform1/RConn1 -- Bushing Joint/RConn1
  Simulink-PS Converter4/RConn1 -- Bushing Joint/LConn6
  Simulink-PS Converter/RConn1 -- Bushing Joint/LConn2
  "{W}"/RConn1 -- Rigid Transform/LConn1
  Rigid Transform/RConn1 -- Bushing Joint/LConn1
  Brick Solid/LConn1 -- Rigid Transform1/LConn1 -- Cartesian Joint/LConn1
  "{F}"/RConn1 -- Cartesian Joint/RConn1

== system stewart_platform_model/Ground/None ==
  d : Inport
  Bus Selector : BusSelector  OutputSignals=D_w
  Terminator : Terminator
  "{W}" : PMIOPort  Side=Left
  "{F}" : PMIOPort  Port=2  Side=Right
  wires:
  d/1 -> Bus Selector/1
  Bus Selector/1 -> Terminator/1  "<D_w>"
  connections:
  "{W}"/RConn1 -- "{F}"/RConn1

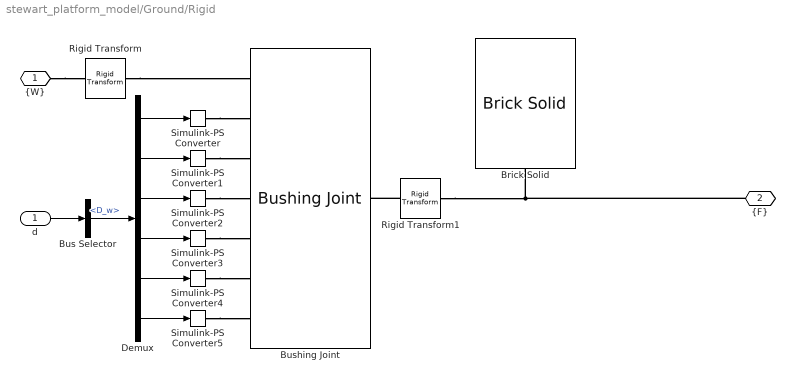
== system stewart_platform_model/Ground/Rigid ==
  d : Inport
  Brick Solid : sm_lib/Body Elements/Brick Solid  GraphicAmbientColor=[0.15 0.15 0.15 1.0]  BasedOnType=Density  BrickDimensions=[0.5 0.5 0.1]  BrickDimensionUnits=m  CenterOfMass=[0 0 0]  CenterOfMassUnits=m  GraphicDiffuseColor=[0.5 0.5 0.5]  Density=1000  DensityUnits=kg/m^3  DoExposeReferenceFrame=off  GraphicEmissiveColor=[0.0 0.0 0.0 1.0]  ExportEntireGeometry=off  SerializedFrames=<Frames><Frame><Id>Frame2</Id><Value><Name>top</Name><Origin><Source>GeometricFeature</Source><FeatureName>+z surface</FeatureName></Origin><PrimaryAxis><DefinedDirection>+Z</DefinedDirection><Source>ReferenceFrame</Source><SourceDirection>+Z</SourceDirection><FeatureName></FeatureName></PrimaryAxis><SecondaryAxis><DefinedDirection>+X</DefinedDirection><Source>ReferenceFrame</Source><SourceDirection>+X</SourceDirection><FeatureName></FeatureName></SecondaryAxis></Value></Frame></Frames>  MarkerShape=Sphere  MarkerSize=10  GraphicType=FromGeometry  InertiaType=CalculateFromGeometry  Mass=1  MassUnits=kg  MomentsOfInertia=[1 1 1]  MomentsOfInertiaUnits=kg*m^2  GraphicOpacity=1.0  ProductsOfInertia=[0 0 0]  ProductsOfInertiaUnits=kg*m^2  GraphicShininess=75  GraphicSpecularColor=[0.5 0.5 0.5 1.0]  GraphicVisPropType=SimpleVisualProperties
  Bus Selector : BusSelector  OutputSignals=D_w
  Bushing Joint : sm_lib/Joints/Bushing Joint  JointMode=Normal  SenseConstraintForce=off  SenseConstraintForceX=off  SenseConstraintForceY=off  SenseConstraintForceZ=off  SenseConstraintTorque=off  SenseConstraintTorqueX=off  SenseConstraintTorqueY=off  SenseConstraintTorqueZ=off  SenseTotalForce=off  SenseTotalForceX=off  SenseTotalForceY=off  SenseTotalForceZ=off  SenseTotalTorque=off  SenseTotalTorqueX=off  SenseTotalTorqueY=off  SenseTotalTorqueZ=off  CompositeWrenchDir=FollowerOnBase  CompositeWrenchFrame=BaseFrame  PxEquilibriumPosition=0  PxEquilibriumPositionUnits=m  PxSpringStiffness=0  PxSpringStiffnessUnits=N/m  PxDampingCoefficient=0  PxDampingCoefficientUnits=N/(m/s)  PxTorqueActuationMode=ComputedTorque  PxMotionActuationMode=InputMotion  PxSensePosition=off  PxSenseVelocity=off  PxSenseAcceleration=off  PxSenseTorqueForce=off  PxSenseLowerLimitTorqueForce=off  PxSenseUpperLimitTorqueForce=off  PxLowerLimitSpecify=off  PxLowerLimitBound=-1  PxLowerLimitBoundUnits=m  PxLowerLimitStiffness=1e6  PxLowerLimitStiffnessUnits=N/m  PxLowerLimitDamping=1e3  PxLowerLimitDampingUnits=N/(m/s)  PxLowerLimitTransitionRegionWidth=1e-4  PxLowerLimitTransitionRegionWidthUnits=m  PxUpperLimitSpecify=off  PxUpperLimitBound=1  PxUpperLimitBoundUnits=m  PxUpperLimitStiffness=1e6  PxUpperLimitStiffnessUnits=N/m  PxUpperLimitDamping=1e3  PxUpperLimitDampingUnits=N/(m/s)  PxUpperLimitTransitionRegionWidth=1e-4  PxUpperLimitTransitionRegionWidthUnits=m  PxPositionTargetSpecify=off  PxPositionTargetPriority=High  PxPositionTargetValue=0  PxPositionTargetValueUnits=m  PxVelocityTargetSpecify=off  PxVelocityTargetPriority=High  PxVelocityTargetValue=0  PxVelocityTargetValueUnits=m/s  PyEquilibriumPosition=0  PyEquilibriumPositionUnits=m  PySpringStiffness=0  PySpringStiffnessUnits=N/m  PyDampingCoefficient=0  PyDampingCoefficientUnits=N/(m/s)  PyTorqueActuationMode=ComputedTorque  PyMotionActuationMode=InputMotion  PySensePosition=off  PySenseVelocity=off  PySenseAcceleration=off  PySenseTorqueForce=off  PySenseLowerLimitTorqueForce=off  PySenseUpperLimitTorqueForce=off  PyLowerLimitSpecify=off  PyLowerLimitBound=-1  PyLowerLimitBoundUnits=m  PyLowerLimitStiffness=1e6  PyLowerLimitStiffnessUnits=N/m  PyLowerLimitDamping=1e3  PyLowerLimitDampingUnits=N/(m/s)  PyLowerLimitTransitionRegionWidth=1e-4  PyLowerLimitTransitionRegionWidthUnits=m  PyUpperLimitSpecify=off  PyUpperLimitBound=1  PyUpperLimitBoundUnits=m  PyUpperLimitStiffness=1e6  PyUpperLimitStiffnessUnits=N/m  PyUpperLimitDamping=1e3  PyUpperLimitDampingUnits=N/(m/s)  PyUpperLimitTransitionRegionWidth=1e-4  PyUpperLimitTransitionRegionWidthUnits=m  PyPositionTargetSpecify=off  PyPositionTargetPriority=High  PyPositionTargetValue=0  PyPositionTargetValueUnits=m  PyVelocityTargetSpecify=off  PyVelocityTargetPriority=High  PyVelocityTargetValue=0  PyVelocityTargetValueUnits=m/s  PzEquilibriumPosition=0  PzEquilibriumPositionUnits=m  PzSpringStiffness=0  PzSpringStiffnessUnits=N/m  PzDampingCoefficient=0  PzDampingCoefficientUnits=N/(m/s)  PzTorqueActuationMode=ComputedTorque  PzMotionActuationMode=InputMotion  PzSensePosition=off  PzSenseVelocity=off  PzSenseAcceleration=off  PzSenseTorqueForce=off  PzSenseLowerLimitTorqueForce=off  PzSenseUpperLimitTorqueForce=off  PzLowerLimitSpecify=off  PzLowerLimitBound=-1  PzLowerLimitBoundUnits=m  PzLowerLimitStiffness=1e6  PzLowerLimitStiffnessUnits=N/m  PzLowerLimitDamping=1e3  PzLowerLimitDampingUnits=N/(m/s)  PzLowerLimitTransitionRegionWidth=1e-4  PzLowerLimitTransitionRegionWidthUnits=m  PzUpperLimitSpecify=off  PzUpperLimitBound=1  PzUpperLimitBoundUnits=m  PzUpperLimitStiffness=1e6  PzUpperLimitStiffnessUnits=N/m  PzUpperLimitDamping=1e3  PzUpperLimitDampingUnits=N/(m/s)  PzUpperLimitTransitionRegionWidth=1e-4  PzUpperLimitTransitionRegionWidthUnits=m  PzPositionTargetSpecify=off  PzPositionTargetPriority=High  PzPositionTargetValue=0  PzPositionTargetValueUnits=m  PzVelocityTargetSpecify=off  PzVelocityTargetPriority=High  PzVelocityTargetValue=0  PzVelocityTargetValueUnits=m/s  RxEquilibriumPosition=0  RxEquilibriumPositionUnits=deg  RxSpringStiffness=0  RxSpringStiffnessUnits=N*m/deg  RxDampingCoefficient=0  RxDampingCoefficientUnits=N*m/(deg/s)  RxTorqueActuationMode=ComputedTorque  RxMotionActuationMode=InputMotion  RxSensePosition=off  RxSenseVelocity=off  RxSenseAcceleration=off  RxSenseTorqueForce=off  RxSenseLowerLimitTorqueForce=off  RxSenseUpperLimitTorqueForce=off  RxLowerLimitSpecify=off  RxLowerLimitBound=-90  RxLowerLimitBoundUnits=deg  RxLowerLimitStiffness=1e4  RxLowerLimitStiffnessUnits=N*m/deg  RxLowerLimitDamping=10  RxLowerLimitDampingUnits=N*m/(deg/s)  RxLowerLimitTransitionRegionWidth=0.1  RxLowerLimitTransitionRegionWidthUnits=deg  RxUpperLimitSpecify=off  RxUpperLimitBound=90  RxUpperLimitBoundUnits=deg  RxUpperLimitStiffness=1e4  RxUpperLimitStiffnessUnits=N*m/deg  RxUpperLimitDamping=10  RxUpperLimitDampingUnits=N*m/(deg/s)  RxUpperLimitTransitionRegionWidth=0.1  RxUpperLimitTransitionRegionWidthUnits=deg  RxPositionTargetSpecify=off  RxPositionTargetPriority=High  RxPositionTargetValue=0  RxPositionTargetValueUnits=deg  RxVelocityTargetSpecify=off  RxVelocityTargetPriority=High  RxVelocityTargetValue=0  RxVelocityTargetValueUnits=deg/s  RyEquilibriumPosition=0  RyEquilibriumPositionUnits=deg  RySpringStiffness=0  RySpringStiffnessUnits=N*m/deg  RyDampingCoefficient=0  RyDampingCoefficientUnits=N*m/(deg/s)  RyTorqueActuationMode=ComputedTorque  RyMotionActuationMode=InputMotion  RySensePosition=off  RySenseVelocity=off  RySenseAcceleration=off  RySenseTorqueForce=off  RySenseLowerLimitTorqueForce=off  RySenseUpperLimitTorqueForce=off  RyLowerLimitSpecify=off  RyLowerLimitBound=-90  RyLowerLimitBoundUnits=deg  RyLowerLimitStiffness=1e4  RyLowerLimitStiffnessUnits=N*m/deg  RyLowerLimitDamping=10  RyLowerLimitDampingUnits=N*m/(deg/s)  RyLowerLimitTransitionRegionWidth=0.1  RyLowerLimitTransitionRegionWidthUnits=deg  RyUpperLimitSpecify=off  RyUpperLimitBound=90  RyUpperLimitBoundUnits=deg  RyUpperLimitStiffness=1e4  RyUpperLimitStiffnessUnits=N*m/deg  RyUpperLimitDamping=10  RyUpperLimitDampingUnits=N*m/(deg/s)  RyUpperLimitTransitionRegionWidth=0.1  RyUpperLimitTransitionRegionWidthUnits=deg  RyPositionTargetSpecify=off  RyPositionTargetPriority=High  RyPositionTargetValue=0  RyPositionTargetValueUnits=deg  RyVelocityTargetSpecify=off  RyVelocityTargetPriority=High  RyVelocityTargetValue=0  RyVelocityTargetValueUnits=deg/s  RzEquilibriumPosition=0  RzEquilibriumPositionUnits=deg  RzSpringStiffness=0  RzSpringStiffnessUnits=N*m/deg  RzDampingCoefficient=0  RzDampingCoefficientUnits=N*m/(deg/s)  RzTorqueActuationMode=ComputedTorque  RzMotionActuationMode=InputMotion  RzSensePosition=off  RzSenseVelocity=off  RzSenseAcceleration=off  RzSenseTorqueForce=off  RzSenseLowerLimitTorqueForce=off  RzSenseUpperLimitTorqueForce=off  RzLowerLimitSpecify=off  RzLowerLimitBound=-90  RzLowerLimitBoundUnits=deg  RzLowerLimitStiffness=1e4  RzLowerLimitStiffnessUnits=N*m/deg  RzLowerLimitDamping=10  RzLowerLimitDampingUnits=N*m/(deg/s)  RzLowerLimitTransitionRegionWidth=0.1  RzLowerLimitTransitionRegionWidthUnits=deg  RzUpperLimitSpecify=off  RzUpperLimitBound=90  RzUpperLimitBoundUnits=deg  RzUpperLimitStiffness=1e4  RzUpperLimitStiffnessUnits=N*m/deg  RzUpperLimitDamping=10  RzUpperLimitDampingUnits=N*m/(deg/s)  RzUpperLimitTransitionRegionWidth=0.1  RzUpperLimitTransitionRegionWidthUnits=deg  RzPositionTargetSpecify=off  RzPositionTargetPriority=High  RzPositionTargetValue=0  RzPositionTargetValueUnits=deg  RzVelocityTargetSpecify=off  RzVelocityTargetPriority=High  RzVelocityTargetValue=0  RzVelocityTargetValueUnits=deg/s
  Demux : Demux  Outputs=6
  Rigid Transform : sm_lib/Frames and Transforms/Rigid Transform  TranslationMethod=Cartesian  TranslationStandardOffset=0  TranslationLengthUnit=m  TranslationStandardAxis=+Z  TranslationCartesianOffset=ground.rot_point  TranslationROffset=0  TranslationROffsetUnits=m  TranslationZOffset=0  TranslationZOffsetUnits=m  TranslationThetaOffset=0  TranslationThetaOffsetUnits=deg  RotationMethod=None  RotationAngleUnits=deg  RotationStandardAxis=+Z  RotationAngle=0.0  RotationArbitraryAxis=[0 0 1]  FollAlignAxisA=+X  BaseAlignAxisA=+Y  FollAlignAxisB=+Y  BaseAlignAxisB=+Z  RotationSequenceAxes=FollowerAxes  RotationSequence=XYX  RotationSequenceAngles=[0 0 0]  RotationSequenceAnglesUnits=deg  RotationMatrix=[1 0 0; 0 1 0; 0 0 1]
  Rigid Transform1 : sm_lib/Frames and Transforms/Rigid Transform  TranslationMethod=Cartesian  TranslationStandardOffset=0  TranslationLengthUnit=m  TranslationStandardAxis=+Z  TranslationCartesianOffset=ground.rot_point  TranslationROffset=0  TranslationROffsetUnits=m  TranslationZOffset=0  TranslationZOffsetUnits=m  TranslationThetaOffset=0  TranslationThetaOffsetUnits=deg  RotationMethod=None  RotationAngleUnits=deg  RotationStandardAxis=+Z  RotationAngle=0.0  RotationArbitraryAxis=[0 0 1]  FollAlignAxisA=+X  BaseAlignAxisA=+Y  FollAlignAxisB=+Y  BaseAlignAxisB=+Z  RotationSequenceAxes=FollowerAxes  RotationSequence=XYX  RotationSequenceAngles=[0 0 0]  RotationSequenceAnglesUnits=deg  RotationMatrix=[1 0 0; 0 1 0; 0 0 1]
  Simulink-PS Converter{,1..5} (6 alike) : nesl_utility/Simulink-PS Converter  PhysicalDomain=network_engine_domain  SubClassName=ps_input  LeftPortType=input  RightPortType=output  PseudoPeriodic=off  Frequencies=[]  NoiseDistribution=none  NoiseParameters=[]  Unit=1  AffineConversion=off  FilteringAndDerivatives=filter  SimscapeFilterOrder=2  InputFilterTimeConstant=0.001  UdotUserProvided=0
  "{W}" : PMIOPort  Side=Left
  "{F}" : PMIOPort  Port=2  Side=Right
  wires:
  d/1 -> Bus Selector/1
  Demux/2 -> Simulink-PS Converter1/1
  Demux/5 -> Simulink-PS Converter4/1
  Demux/3 -> Simulink-PS Converter2/1
  Demux/4 -> Simulink-PS Converter3/1
  Demux/6 -> Simulink-PS Converter5/1
  Demux/1 -> Simulink-PS Converter/1
  Bus Selector/1 -> Demux/1  "<D_w>"
  connections:
  Simulink-PS Converter1/RConn1 -- Bushing Joint/LConn3
  Simulink-PS Converter3/RConn1 -- Bushing Joint/LConn5
  Simulink-PS Converter4/RConn1 -- Bushing Joint/LConn6
  Simulink-PS Converter5/RConn1 -- Bushing Joint/LConn7
  Simulink-PS Converter/RConn1 -- Bushing Joint/LConn2
  Simulink-PS Converter2/RConn1 -- Bushing Joint/LConn4
  Rigid Transform/RConn1 -- Bushing Joint/LConn1
  "{W}"/RConn1 -- Rigid Transform/LConn1
  Rigid Transform1/RConn1 -- Bushing Joint/RConn1
  Rigid Transform1/LConn1 -- "{F}"/RConn1 -- Brick Solid/LConn1
